simulink model "demo_overlap"  (R2026a)
settings: Solver=FixedStepDiscrete  StopTime=2  FixedStep=.1
settings Model: Creator=harry_31916  LastModifiedBy=harry_31916

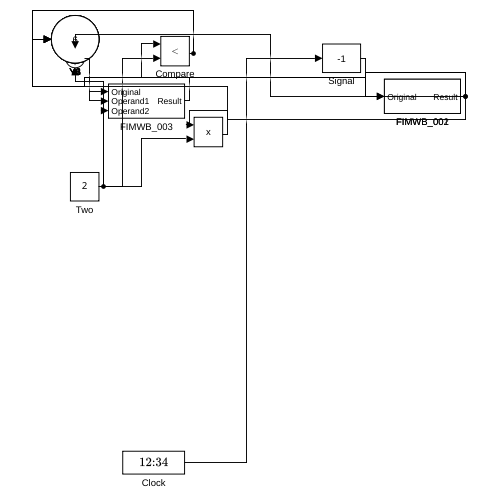
[thumbnail: Simulink's stored preview of the top-level diagram]
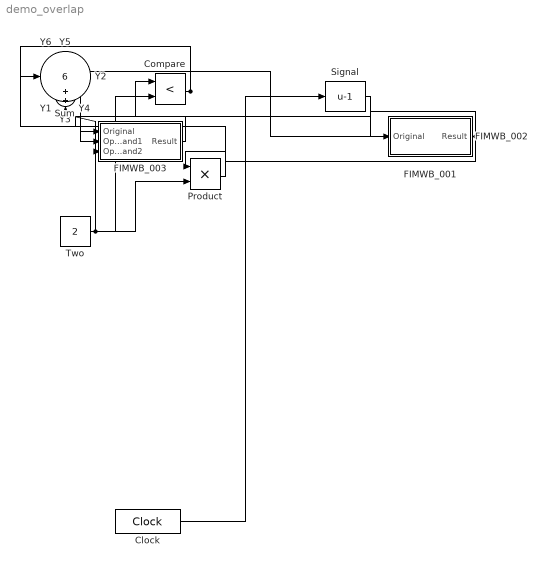
== system demo_overlap ==
  Clock : DigitalClock  SampleTime=.1
  Compare : RelationalOperator  Operator=<  OutDataTypeStr=boolean  RndMeth=Simplest  InputSameDT=off
  FIMWB_001 : Subsystem  Tag=fimwb.fault.1
  FIMWB_002 : Subsystem  Tag=fimwb.fault.2
  FIMWB_003 : Subsystem  Tag=fimwb.fault.3
  Product : Product  Inputs=**
  Signal : Bias  Bias=-1  SaturateOnIntegerOverflow=off
  Sum : Sum
  Two : Constant  Value=2
  Y1 : Outport  SampleTime=0.1
  Y2 : Outport  Port=2  SampleTime=0.1
  Y3 : Outport  Port=3  SampleTime=0.1
  Y4 : Outport  Port=4  SampleTime=0.1
  Y5 : Outport  Port=5  SampleTime=0.1
  Y6 : Outport  Port=6  SampleTime=0.1
  wires:
  Clock/1 -> Signal/1
  Two/1 -> Sum/2, Product/2, Compare/2, FIMWB_003/3(Operand2)
  Product/1 -> Y4/1
  Compare/1 -> Y5/1, Y6/1
  Sum/1 -> FIMWB_003/1(Original)
  FIMWB_003/1(Result) -> Y3/1
  Signal/1 -> FIMWB_002/1(Original)
  FIMWB_002/1(Result) -> Product/1, Compare/1, Y1/1, Y2/1, FIMWB_001/1(Original)
  FIMWB_001/1(Result) -> Sum/1, FIMWB_003/2(Operand1)

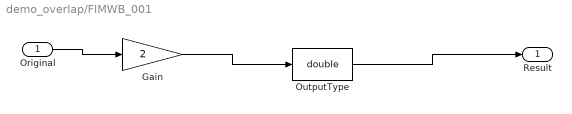
== system demo_overlap/FIMWB_001 ==
  Original : Inport
  Gain : Gain  Gain=2  OutDataTypeStr=Inherit: Same as input
  OutputType : DataTypeConversion  OutDataTypeStr=double  RndMeth=Round
  Result : Outport
  wires:
  Original/1 -> Gain/1
  Gain/1 -> OutputType/1
  OutputType/1 -> Result/1

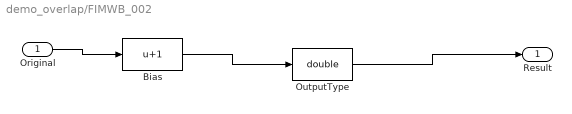
== system demo_overlap/FIMWB_002 ==
  Original : Inport
  Bias : Bias  Bias=1  SaturateOnIntegerOverflow=off
  OutputType : DataTypeConversion  OutDataTypeStr=double  RndMeth=Round
  Result : Outport
  wires:
  Original/1 -> Bias/1
  Bias/1 -> OutputType/1
  OutputType/1 -> Result/1

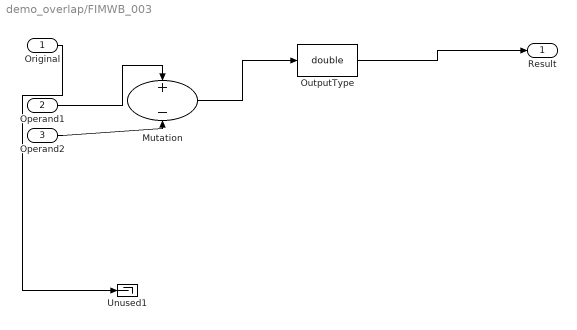
== system demo_overlap/FIMWB_003 ==
  Original : Inport
  Operand1 : Inport  Port=2
  Operand2 : Inport  Port=3
  Mutation : Sum  Inputs=+-
  OutputType : DataTypeConversion  OutDataTypeStr=double  RndMeth=Round
  Unused1 : Terminator
  Result : Outport
  wires:
  Operand1/1 -> Mutation/1
  Operand2/1 -> Mutation/2
  Mutation/1 -> OutputType/1
  OutputType/1 -> Result/1
  Original/1 -> Unused1/1
